simulink model "GK"  (R2024b)
settings: Solver=FixedStepAuto  StartTime=0.0  StopTime=10.0  RelTol=1e-3
undefined symbols (not defined in the file): FRKAP
settings Model: Creator=Student  LastModifiedBy=Student
settings DataIOCC: SaveFormat=Array
settings OptimizationCC: DefaultParameterBehavior=Inlined  EnhancedBackFolding=on  PassReuseOutputArgsAs=Individual arguments  ZeroExternalMemoryAtStartup=off  ZeroInternalMemoryAtStartup=off  OptimizeBlockOrder=speed  DifferentSizesBufferReuse=on  OptimizationCustomize=off  EfficientTunableParamExpr=on
settings DebuggingCC: ParameterTunabilityLossMsg=error
settings HardwareCC: ProdLongLongMode=on
settings ModelReferenceCC: EnableRefExpFcnMdlSchedulingChecks=on
settings SFSimCC: MATLABDynamicMemAlloc=off
settings RTWCC: Description=Embedded Coder  SystemTargetFile=ert.tlc  TemplateMakefile=ert_default_tmf  GPUComputeCapability=3.5
settings CodeAppCC: ForceParamTrailComments=on  IgnoreCustomStorageClasses=off  OperatorAnnotations=on  SimulinkDataObjDesc=on  SFDataObjDesc=on  InsertBlockDesc=on
settings ERTTargetCC: TargetLangStandard=C99 (ISO)  GenerateSampleERTMain=on  ERTCustomFileTemplate=example_file_process.tlc  DynamicArrayContainerType=coder::array

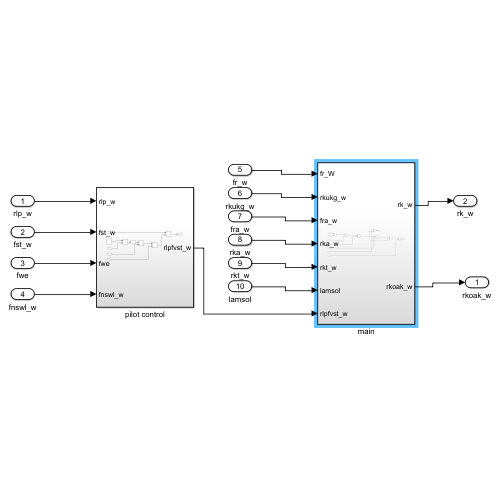
[thumbnail: Simulink's stored preview of the top-level diagram]
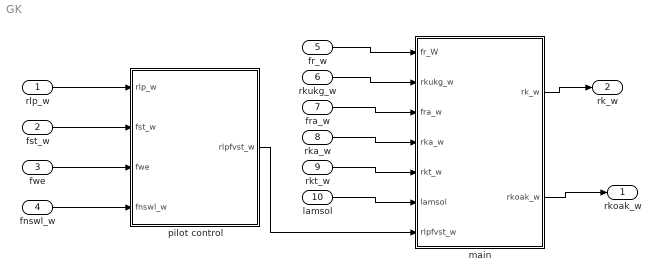
== system GK ==
  rlp_w : Inport
  fst_w : Inport  Port=2
  fwe : Inport  Port=3
  fnswl_w : Inport  Port=4
  fr_w : Inport  Port=5
  rkukg_w : Inport  Port=6
  fra_w : Inport  Port=7
  rka_w : Inport  Port=8
  rkt_w : Inport  Port=9
  lamsol : Inport  Port=10
  main : Subsystem
  pilot control : Subsystem
  rkoak_w : Outport
  rk_w : Outport  Port=2
  wires:
  fwe/1 -> pilot control/3(fwe)
  fnswl_w/1 -> pilot control/4(fnswl_w)
  fr_w/1 -> main/1(fr_W)
  rkukg_w/1 -> main/2(rkukg_w)
  fra_w/1 -> main/3(fra_w)
  rka_w/1 -> main/4(rka_w)
  lamsol/1 -> main/6(lamsol)
  rkt_w/1 -> main/5(rkt_w)
  rlp_w/1 -> pilot control/1(rlp_w)
  fst_w/1 -> pilot control/2(fst_w)
  main/1(rk_w) -> rk_w/1
  main/2(rkoak_w) -> rkoak_w/1
  pilot control/1(rlpfvst_w) -> main/7(rlpfvst_w)

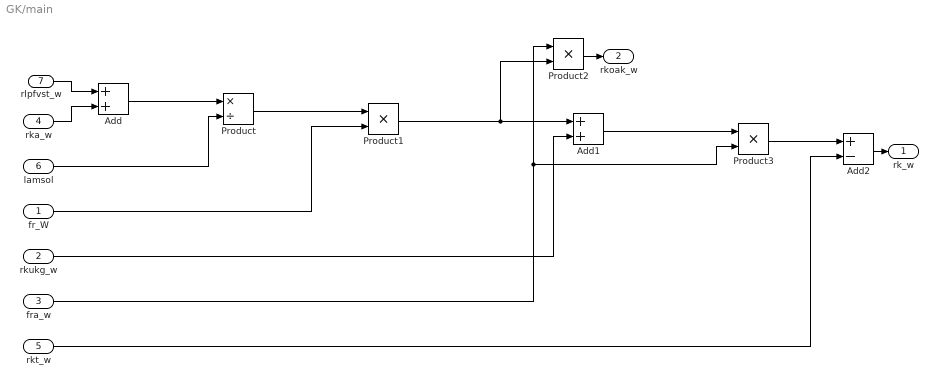
== system GK/main ==
  fr_W : Inport  OutMin=[0]  OutMax=[1.99997]  OutDataTypeStr=fixdt(0,16,1/32768,0)
  rkukg_w : Inport  Port=2  OutMin=[0]  OutMax=[3071.95]  OutDataTypeStr=fixdt(0,16,3/64,0)
  fra_w : Inport  Port=3  OutMin=[0]  OutMax=[1.99997]  OutDataTypeStr=fixdt(0,16,1/32768,0)
  rka_w : Inport  Port=4  OutMin=[0]  OutMax=[3071.95]  OutDataTypeStr=fixdt(0,16,3/64,0)
  rkt_w : Inport  Port=5  OutMin=[0]  OutMax=[3071.95]  OutDataTypeStr=fixdt(0,16,3/64,0)
  lamsol : Inport  Port=6  OutMin=[0]  OutMax=[15.999]  OutDataTypeStr=fixdt(0,16,1/4096,0)
  rlpfvst_w : Inport  Port=7  OutMin=[0]  OutMax=[3071.95]  OutDataTypeStr=fixdt(0,16,3/64,0)  LockScale=on
  Add : Sum  OutDataTypeStr=uint16  AccumDataTypeStr=uint16  SaturateOnIntegerOverflow=on
  Add1 : Sum  OutDataTypeStr=uint16  AccumDataTypeStr=uint16  SaturateOnIntegerOverflow=on
  Add2 : Sum  Inputs=+-  OutMin=[0]  OutMax=[3071.95]  OutDataTypeStr=fixdt(0,16,3/64,0)  SaturateOnIntegerOverflow=on  LockScale=on
  Product : Product  Inputs=*/  OutDataTypeStr=uint16  SaturateOnIntegerOverflow=on
  Product1 : Product  OutDataTypeStr=uint16  SaturateOnIntegerOverflow=on
  Product2 : Product  OutMin=[0]  OutMax=[3071.95]  OutDataTypeStr=fixdt(0,16,3/64,0)  SaturateOnIntegerOverflow=on  LockScale=on
  Product3 : Product  OutDataTypeStr=uint16  SaturateOnIntegerOverflow=on
  rk_w : Outport  OutMin=[0]  OutMax=[3071.95]  OutDataTypeStr=fixdt(0,16,3/64,0)
  rkoak_w : Outport  Port=2  OutMin=[0]  OutMax=[3071.95]  OutDataTypeStr=fixdt(0,16,3/64,0)
  wires:
  Product1/1 -> Add1/1, Product2/2
  Add1/1 -> Product3/1
  Product/1 -> Product1/1
  lamsol/1 -> Product/2
  fra_w/1 -> Product3/2, Product2/1
  fr_W/1 -> Product1/2
  rka_w/1 -> Add/2
  rkukg_w/1 -> Add1/2
  Add2/1 -> rk_w/1
  Product3/1 -> Add2/1
  rkt_w/1 -> Add2/2
  Product2/1 -> rkoak_w/1
  Add/1 -> Product/1
  rlpfvst_w/1 -> Add/1

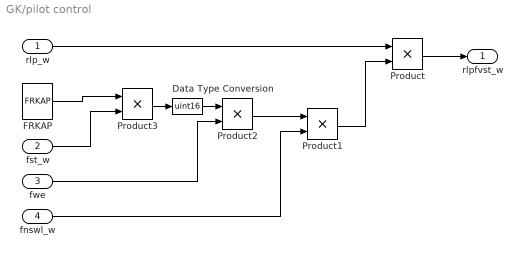
== system GK/pilot control ==
  rlp_w : Inport  OutMin=[0]  OutMax=[1535.98]  OutDataTypeStr=fixdt(0,16,3/128,0)  LockScale=on
  fst_w : Inport  Port=2  OutMin=[0]  OutMax=[63.999]  OutDataTypeStr=fixdt(0,16,1/1024,0)
  fwe : Inport  Port=3  OutMin=[0]  OutMax=[1.99219]  OutDataTypeStr=fixdt(0,8,1/128,0)
  fnswl_w : Inport  Port=4  OutMin=[0]  OutMax=[16]  OutDataTypeStr=fixdt(0,16,2/4096,0)
  Data Type Conversion : DataTypeConversion  OutDataTypeStr=uint16  RndMeth=Floor
  FRKAP : Constant  Value=FRKAP  OutMin=[0]  OutMax=[1.99219]
  Product : Product  OutMin=[0]  OutMax=[3071.95]  OutDataTypeStr=fixdt(0,16,3/64,0)  SaturateOnIntegerOverflow=on
  Product1 : Product  OutDataTypeStr=uint16  SaturateOnIntegerOverflow=on
  Product2 : Product  OutDataTypeStr=uint16  SaturateOnIntegerOverflow=on
  Product3 : Product  SaturateOnIntegerOverflow=on
  rlpfvst_w : Outport  OutMin=[0]  OutMax=[3071.95]  OutDataTypeStr=fixdt(0,16,3/64,0)  LockScale=on
  wires:
  FRKAP/1 -> Product3/1
  rlp_w/1 -> Product/1
  Product2/1 -> Product1/1
  Product1/1 -> Product/2
  Product/1 -> rlpfvst_w/1
  fnswl_w/1 -> Product1/2
  fwe/1 -> Product2/2
  fst_w/1 -> Product3/2
  Product3/1 -> Data Type Conversion/1
  Data Type Conversion/1 -> Product2/1
